simulink model "Template_v5_0_0_2026a_Linear"  (R2026a)
settings: Solver=ode4  StopTime=tsim  FixedStep=baseRate  RelTol=1e-6  AbsTol=1e-6
PreLoadFcn:
  | spot.buses.define;
  | if ~exist('simMode', 'var'), simMode = 1; end
InitFcn:
  | spot.buses.define;
  | if ~exist('simMode', 'var'), simMode = 1; end
values from neighbouring files (symbols this model uses):
  customControllerParamsBLACK = struct('unused', 0)    [SPOT_User_Parameters.m]
  customControllerParamsBLUE = struct('unused', 0)    [SPOT_User_Parameters.m]
  customControllerParamsRED = struct('unused', 0)    [SPOT_User_Parameters.m]
  customPlannerParamsBLACK = struct('unused', 0)    [SPOT_User_Parameters.m]
  customPlannerParamsBLUE = struct('unused', 0)    [SPOT_User_Parameters.m]
  customPlannerParamsRED = struct('unused', 0)    [SPOT_User_Parameters.m]
undefined symbols (not defined in the file or in its folder): baseRate, BLACK, BLUE, dataRate, DiscIntNeverNeededParam, F_thrusters_BLACK, F_thrusters_BLUE, F_thrusters_RED, home_states_BLACK, home_states_BLUE, home_states_RED, IBLACK, IBLUE, init_states_BLACK, init_states_BLUE, init_states_RED, IRED, K_BLACK, K_BLUE, K_RED, mBLACK, mBLUE, mRED, phase, Phase0_End, Phase1_End, Phase2_End, Phase3_End, Phase4_End, Phase5_End, PWMFreq, RED, tableDamping_BLACK, tableDamping_BLUE, tableDamping_RED, tableSlope, thrust_decay_BLACK, thrust_decay_BLUE, thrust_decay_RED, thruster_dist2CG_BLACK, thruster_dist2CG_BLUE, thruster_dist2CG_RED, time, xLength, yLength
libraries: nvidiaCommlib x1
(part 1 of 2)
settings Model: Creator=SPOT  LastModifiedBy=alexandercrain
settings OptimizationCC: MaxStackSize=200000
settings HardwareCC: ProdBitPerLong=64.0  ProdLargestAtomicInteger=LongLong  ProdLargestAtomicFloat=Double  ProdHWDeviceType=ARM Compatible->ARM Cortex-A (64-bit)
settings RTWCC: SystemTargetFile=ert.tlc  HardwareBoard=NVIDIA Jetson  TLCOptions="-aInlineSetEventsForThisBaseRateFcn=TLC_FALSE -aSuppressMultiTaskScheduler=TLC_FALSE  -aRateBasedStepFcn=0"  TargetLang=C++  Description=Embedded Coder
settings ERTTargetCC: ExtModeTransport=2.0  DynamicArrayContainerType=coder::array  SupportContinuousTime=on  SupportVariableSizeSignals=on
settings SimscapeCC: SimscapeNominalValues="[{\"value\":\"1\",\"unit\":\"A\"},{\"value\":\"1\",\"unit\":\"bar\"},{\"value\":\"1\",\"unit\":\"cm^2\"},{\"value\":\"1\",\"unit\":\"cm^3/s\"},{\"value\":\"1\",\"unit\":\"kJ/kg\"},{\"value\":\"1\",\"unit\":\"kW\"},{\"value\":\"1\",\"unit\":\"l\"},{\"value\":\"1\",\"unit\":\"N\"},{\"value\":\"1\",\"unit\":\"N*m\"},{\"value\":\"1\",\"unit\":\"V\"}]"  SimscapeLogType=none  SimscapeLogDataHistory=5000.0

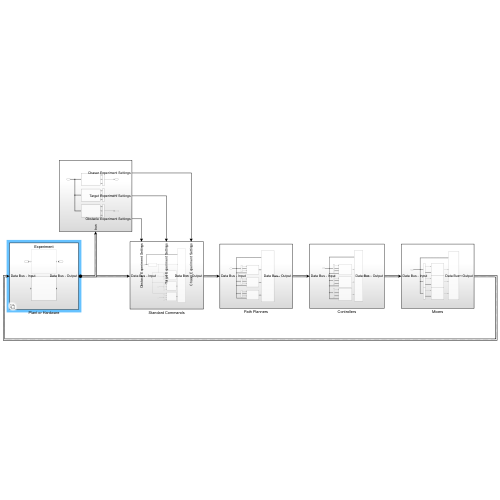
[thumbnail: Simulink's stored preview of the top-level diagram]
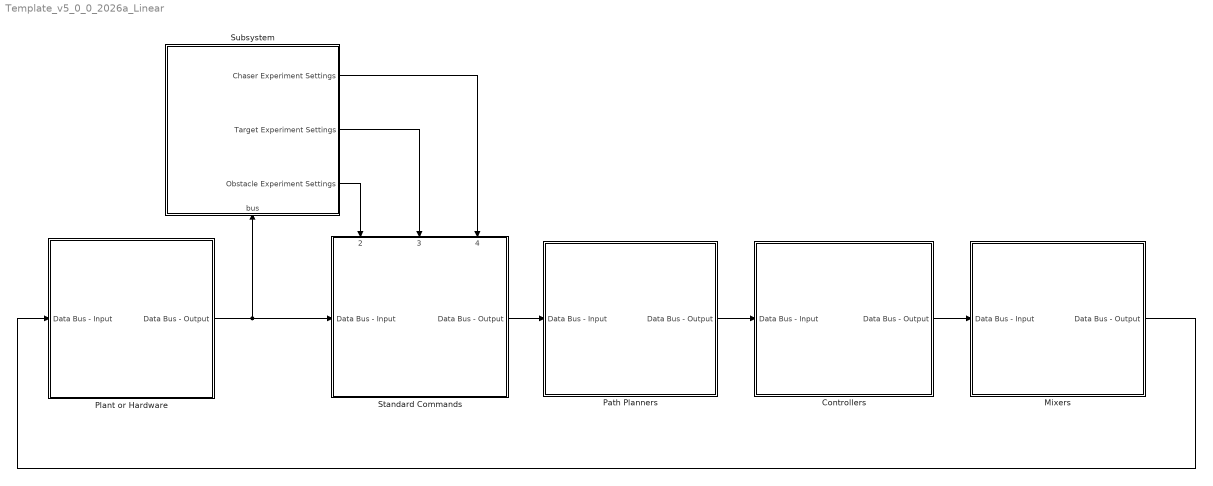
== system Template_v5_0_0_2026a_Linear ==
  Controllers : Subsystem
  Mixers : Subsystem
  Path Planners : Subsystem
  Plant or Hardware : Subsystem  Variant=on
  Standard Commands : Subsystem
      settings: PortSchema="{\"entries\":[{\"content\":{\"sides\":[{\"content\":{\"connectorIds\":[\"In1\"]},\"type\":\"ConnectorPlacement.EquallySpacedRectSide\",\"uuid\":\"35410a40-2c60-43fd-b064-79213576ed15\"},{\"content\":{\"connectorIds\":[\"Out1\"],\"side\":\"RIGHT\"},\"type\":\"ConnectorPlacement.EquallySpacedRectSide\",\"uuid\":\"393452b1-0693-434c-a64d-f21c96477400\"},{\"content\":{\"connectorIds\":[\"In2\",\"In3\",\"In4\"],\"side\":\"TOP\"},\"type\":\"ConnectorPlacement.EquallySpacedRectSide\",\"uuid\":\"b58be7cb-bf37-4612-971a-2054817b9ba4\"}]},\"type\":\"ConnectorPlacement.EquallySpacedConnector\",\"uuid\":\"cc986e65-98fa-43c9-b0c9-e9ff3e868710\"}],\"packageUris\":[\"http://schema.mathworks.com/mf0/Connector/R2020b\"],\"version\":\"1.0\"}"
  Subsystem : Subsystem
      settings: PortSchema="{\"entries\":[{\"content\":{\"sides\":[{\"content\":{},\"type\":\"ConnectorPlacement.EquallySpacedRectSide\",\"uuid\":\"3090d7f9-dd57-46ab-859b-619e032fcf1c\"},{\"content\":{\"connectorIds\":[\"Out1\",\"Out2\",\"Out3\"],\"side\":\"RIGHT\"},\"type\":\"ConnectorPlacement.EquallySpacedRectSide\",\"uuid\":\"1117e6ec-3262-4fcf-b5fe-08b02e10350e\"},{\"content\":{\"side\":\"TOP\"},\"type\":\"ConnectorPlacement.EquallySpacedRectSide\",\"uuid\":\"04f55234-f904-4f76-beb8-0b46031da363\"},{\"content\":{\"connectorIds\":[\"In1\"],\"side\":\"BOTTOM\"},\"type\":\"ConnectorPlacement.EquallySpacedRectSide\",\"uuid\":\"23d719f6-9ee1-4138-a3cc-61c2603cab92\"}]},\"type\":\"ConnectorPlacement.EquallySpacedConnector\",\"uuid\":\"bfffa1a7-ac7c-4cf9-962a-343a4a46f1db\"}],\"packageUris\":[\"http://schema.mathworks.com/mf0/Connector/R2020b\"],\"version\":\"1.0\"}"
  wires:
  Standard Commands/1(Data Bus - Output) -> Path Planners/1(Data Bus - Input)
  Path Planners/1(Data Bus - Output) -> Controllers/1(Data Bus - Input)
  Controllers/1(Data Bus - Output) -> Mixers/1(Data Bus - Input)
  Subsystem/1(Chaser Experiment Settings) -> Standard Commands/4(Chaser Experiment Settings)
  Subsystem/2(Target Experiment Settings) -> Standard Commands/3(Target Experiment Settings)
  Subsystem/3(Obstacle Experiment Settings) -> Standard Commands/2(Obstacle Experiment Settings)
  Mixers/1(Data Bus - Output) -> Plant or Hardware/1(Data Bus - Input)
  Plant or Hardware/1(Data Bus - Output) -> Standard Commands/1(Data Bus - Input), Subsystem/1(bus)

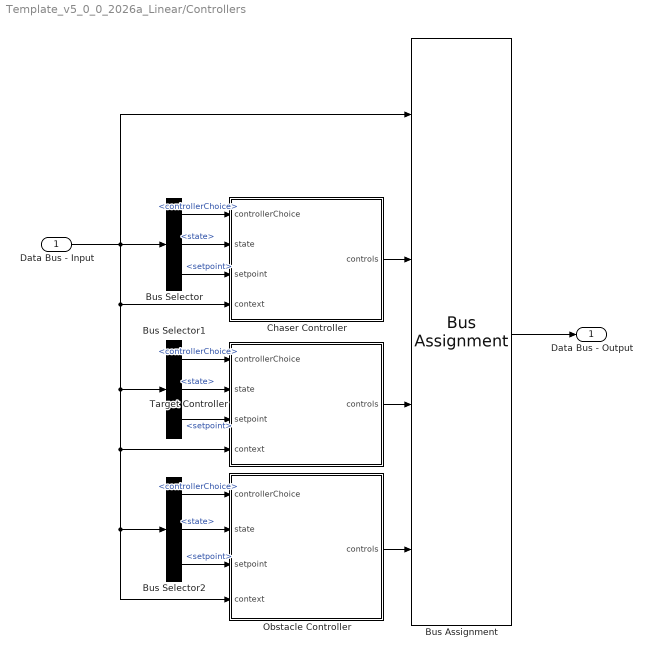
== system Template_v5_0_0_2026a_Linear/Controllers ==
  Data Bus - Input : Inport  OutDataTypeStr=Bus: SpotBus
  Bus Assignment : BusAssignment  AssignedSignals=RED.controls,BLACK.controls,BLUE.controls
  Bus Selector : BusSelector  OutputSignals=RED.command.controllerChoice,RED.state,RED.setpoint
  Bus Selector1 : BusSelector  OutputSignals=BLACK.command.controllerChoice,BLACK.state,BLACK.setpoint
  Bus Selector2 : BusSelector  OutputSignals=BLUE.command.controllerChoice,BLUE.state,BLUE.setpoint
  Chaser Controller : Subsystem  mask{K=K_RED, customParams=customControllerParamsRED}
      mask prompts: K "LQR Gain Matrix"; customParams "Custom Parameters Struct"
  Obstacle Controller : Subsystem  mask{K=K_BLUE, customParams=customControllerParamsBLUE}
      mask prompts: K "LQR Gain Matrix"; customParams "Custom Parameters Struct"
  Target Controller : Subsystem  mask{K=K_BLACK, customParams=customControllerParamsBLACK}
      mask prompts: K "LQR Gain Matrix"; customParams "Custom Parameters Struct"
  Data Bus - Output : Outport  OutDataTypeStr=Bus: SpotBus
  wires:
  Data Bus - Input/1 -> Bus Assignment/1, Target Controller/4(context), Obstacle Controller/4(context), Bus Selector2/1, Bus Selector1/1, Chaser Controller/4(context), Bus Selector/1
  Bus Selector/1 -> Chaser Controller/1(controllerChoice)  "<controllerChoice>"
  Bus Selector1/1 -> Target Controller/1(controllerChoice)  "<controllerChoice>"
  Bus Selector1/2 -> Target Controller/2(state)  "<state>"
  Bus Selector1/3 -> Target Controller/3(setpoint)  "<setpoint>"
  Bus Selector/2 -> Chaser Controller/2(state)  "<state>"
  Bus Selector/3 -> Chaser Controller/3(setpoint)  "<setpoint>"
  Bus Selector2/1 -> Obstacle Controller/1(controllerChoice)  "<controllerChoice>"
  Bus Selector2/2 -> Obstacle Controller/2(state)  "<state>"
  Bus Selector2/3 -> Obstacle Controller/3(setpoint)  "<setpoint>"
  Chaser Controller/1(controls) -> Bus Assignment/2
  Target Controller/1(controls) -> Bus Assignment/3
  Obstacle Controller/1(controls) -> Bus Assignment/4
  Bus Assignment/1 -> Data Bus - Output/1

== system Template_v5_0_0_2026a_Linear/Mixers ==
  Data Bus - Input : Inport  OutDataTypeStr=Bus: SpotBus
  Bus Assignment : BusAssignment  AssignedSignals=RED.duty,BLACK.duty,BLUE.duty
  Bus Selector : BusSelector  OutputSignals=RED.controls,RED.state
  Bus Selector1 : BusSelector  OutputSignals=BLACK.controls,BLACK.state
  Bus Selector2 : BusSelector  OutputSignals=BLUE.controls,BLUE.state
  Chaser Mixer : Subsystem  mask{thrusterDist=thruster_dist2CG_RED, thrust=F_thrusters_RED, decayPerValve=thrust_decay_RED}
      mask prompts: thrusterDist "Thruster Distances from CG"; thrust "Nominal Force per Thruster"; decayPerValve "Decay per Thruster"
  Obstacle Mixer : Subsystem  mask{thrusterDist=thruster_dist2CG_BLUE, thrust=F_thrusters_BLUE, decayPerValve=thrust_decay_BLUE}
      mask prompts: thrusterDist "Thruster Distances from CG"; thrust "Nominal Force per Thruster"; decayPerValve "Decay per Thruster"
  Target Mixer : Subsystem  mask{thrusterDist=thruster_dist2CG_BLACK, thrust=F_thrusters_BLACK, decayPerValve=thrust_decay_BLACK}
      mask prompts: thrusterDist "Thruster Distances from CG"; thrust "Nominal Force per Thruster"; decayPerValve "Decay per Thruster"
  Data Bus - Output : Outport  OutDataTypeStr=Bus: SpotBus
  wires:
  Data Bus - Input/1 -> Bus Selector2/1, Bus Selector1/1, Bus Assignment/1, Bus Selector/1
  Bus Selector/1 -> Chaser Mixer/1(controls)  "<controls>"
  Bus Selector/2 -> Chaser Mixer/2(state)  "<state>"
  Bus Selector2/1 -> Obstacle Mixer/1(controls)  "<controls>"
  Bus Selector1/1 -> Target Mixer/1(controls)  "<controls>"
  Bus Selector1/2 -> Target Mixer/2(state)  "<state>"
  Bus Selector2/2 -> Obstacle Mixer/2(state)  "<state>"
  Bus Assignment/1 -> Data Bus - Output/1
  Chaser Mixer/1(duty) -> Bus Assignment/2
  Target Mixer/1(duty) -> Bus Assignment/3
  Obstacle Mixer/1(duty) -> Bus Assignment/4

== system Template_v5_0_0_2026a_Linear/Path Planners ==
  Data Bus - Input : Inport  OutDataTypeStr=Bus: SpotBus
  Bus Assignment : BusAssignment  AssignedSignals=RED.setpoint,BLACK.setpoint,BLUE.setpoint
  Bus Selector : BusSelector  OutputSignals=RED.command.plannerChoice,RED.state,RED.command.goal
  Bus Selector1 : BusSelector  OutputSignals=BLACK.command.plannerChoice,BLACK.state,BLACK.command.goal
  Bus Selector2 : BusSelector  OutputSignals=BLUE.command.plannerChoice,BLUE.state,BLUE.command.goal
  Chaser Planner : Subsystem  mask{maxSpeed=0.05, maxTurnRate=0.09, horizon=2, customParams=customPlannerParamsRED, initialPose=init_states_RED}
      mask prompts: maxSpeed "Cruising Speed"; maxTurnRate "Cruising Turn Rate"; horizon "Setpoint Distance"; customParams "User Parameters"; initialPose "Initial Pose"
  Obstacle Planner : Subsystem  mask{maxSpeed=0.05, maxTurnRate=0.09, horizon=2, customParams=customPlannerParamsBLUE, initialPose=init_states_BLUE}
      mask prompts: maxSpeed "Cruising Speed"; maxTurnRate "Cruising Turn Rate"; horizon "Setpoint Distance"; customParams "User Parameters"; initialPose "Initial Pose"
  Target Planner : Subsystem  mask{maxSpeed=0.05, maxTurnRate=0.09, horizon=2, customParams=customPlannerParamsBLACK, initialPose=init_states_BLACK}
      mask prompts: maxSpeed "Cruising Speed"; maxTurnRate "Cruising Turn Rate"; horizon "Setpoint Distance"; customParams "User Parameters"; initialPose "Initial Pose"
  Data Bus - Output : Outport  OutDataTypeStr=Bus: SpotBus
  wires:
  Data Bus - Input/1 -> Chaser Planner/4(context), Target Planner/4(context), Obstacle Planner/4(context), Bus Selector2/1, Bus Selector1/1, Bus Assignment/1, Bus Selector/1
  Chaser Planner/1(setpoint) -> Bus Assignment/2
  Target Planner/1(setpoint) -> Bus Assignment/3
  Obstacle Planner/1(setpoint) -> Bus Assignment/4
  Bus Assignment/1 -> Data Bus - Output/1
  Bus Selector/3 -> Chaser Planner/3(goal)  "<goal>"
  Bus Selector/2 -> Chaser Planner/2(state)  "<state>"
  Bus Selector/1 -> Chaser Planner/1(plannerChoice)  "<plannerChoice>"
  Bus Selector1/1 -> Target Planner/1(plannerChoice)  "<plannerChoice>"
  Bus Selector1/2 -> Target Planner/2(state)  "<state>"
  Bus Selector1/3 -> Target Planner/3(goal)  "<goal>"
  Bus Selector2/1 -> Obstacle Planner/1(plannerChoice)  "<plannerChoice>"
  Bus Selector2/2 -> Obstacle Planner/2(state)  "<state>"
  Bus Selector2/3 -> Obstacle Planner/3(goal)  "<goal>"

== system Template_v5_0_0_2026a_Linear/Plant or Hardware ==
  Data Bus - Input : Inport
  Experiment : Subsystem  VariantControl=simMode == 0
  Simulation : Subsystem  VariantControl=simMode == 1
  Data Bus - Output : Outport

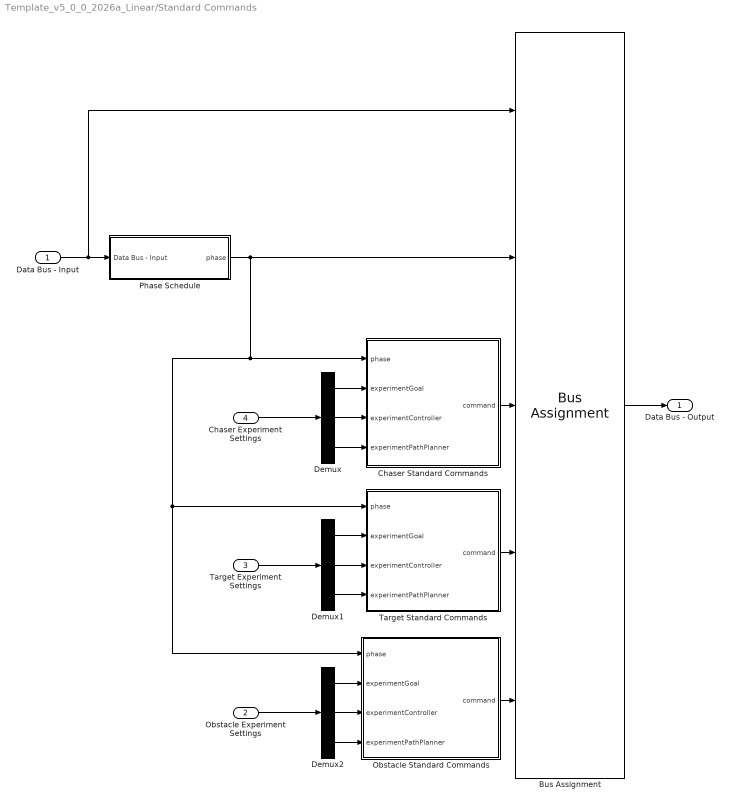
== system Template_v5_0_0_2026a_Linear/Standard Commands ==
  Data Bus - Input : Inport  OutDataTypeStr=Bus: SpotBus
  Obstacle Experiment Settings : Inport  Port=2
  Target Experiment Settings : Inport  Port=3
  Chaser Experiment Settings : Inport  Port=4
  Bus Assignment : BusAssignment  AssignedSignals=phase,RED.command,BLACK.command,BLUE.command
  Chaser Standard Commands : Subsystem  mask{initialPose=init_states_RED, homePose=home_states_RED}
      mask prompts: initialPose "Initial Pose"; homePose "Home Pose"
  Demux : Demux  Outputs=[3,1,1]
  Demux1 : Demux  Outputs=[3,1,1]
  Demux2 : Demux  Outputs=[3,1,1]
  Obstacle Standard Commands : Subsystem  mask{initialPose=init_states_BLUE, homePose=home_states_BLUE}
      mask prompts: initialPose "Initial Pose"; homePose "Home Pose"
  Phase Schedule : Subsystem
  Target Standard Commands : Subsystem  mask{initialPose=init_states_BLACK, homePose=home_states_BLACK}
      mask prompts: initialPose "Initial Pose"; homePose "Home Pose"
  Data Bus - Output : Outport  OutDataTypeStr=Bus: SpotBus
  wires:
  Phase Schedule/1(phase) -> Bus Assignment/2, Chaser Standard Commands/1(phase), Target Standard Commands/1(phase), Obstacle Standard Commands/1(phase)
  Data Bus - Input/1 -> Bus Assignment/1, Phase Schedule/1(Data Bus - Input)
  Chaser Standard Commands/1(command) -> Bus Assignment/3
  Target Standard Commands/1(command) -> Bus Assignment/4
  Obstacle Standard Commands/1(command) -> Bus Assignment/5
  Bus Assignment/1 -> Data Bus - Output/1
  Demux/1 -> Chaser Standard Commands/2(experimentGoal)
  Demux/2 -> Chaser Standard Commands/3(experimentController)
  Demux/3 -> Chaser Standard Commands/4(experimentPathPlanner)
  Chaser Experiment Settings/1 -> Demux/1
  Demux1/1 -> Target Standard Commands/2(experimentGoal)
  Demux1/2 -> Target Standard Commands/3(experimentController)
  Demux1/3 -> Target Standard Commands/4(experimentPathPlanner)
  Target Experiment Settings/1 -> Demux1/1
  Demux2/1 -> Obstacle Standard Commands/2(experimentGoal)
  Demux2/2 -> Obstacle Standard Commands/3(experimentController)
  Demux2/3 -> Obstacle Standard Commands/4(experimentPathPlanner)
  Obstacle Experiment Settings/1 -> Demux2/1

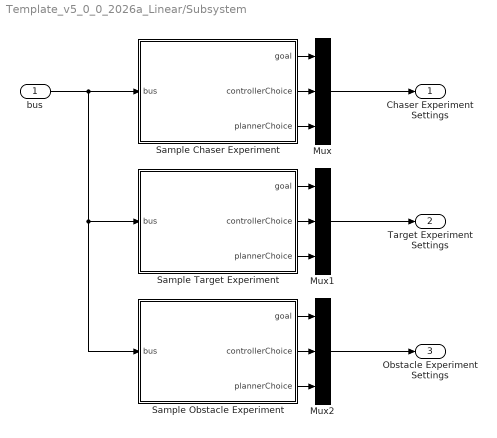
== system Template_v5_0_0_2026a_Linear/Subsystem ==
  bus : Inport  OutDataTypeStr=Bus: SpotBus
  Mux : Mux  Inputs=3
  Mux1 : Mux  Inputs=3
  Mux2 : Mux  Inputs=3
  Sample Chaser Experiment : MATLAB Function  TreatAsAtomicUnit=on
  Sample Obstacle Experiment : MATLAB Function  TreatAsAtomicUnit=on
  Sample Target Experiment : MATLAB Function  TreatAsAtomicUnit=on
  Chaser Experiment Settings : Outport
  Target Experiment Settings : Outport  Port=2
  Obstacle Experiment Settings : Outport  Port=3
  wires:
  bus/1 -> Sample Obstacle Experiment/1(bus), Sample Target Experiment/1(bus), Sample Chaser Experiment/1(bus)
  Sample Chaser Experiment/1(goal) -> Mux/1
  Sample Chaser Experiment/2(controllerChoice) -> Mux/2
  Sample Chaser Experiment/3(plannerChoice) -> Mux/3
  Sample Target Experiment/1(goal) -> Mux1/1
  Sample Target Experiment/2(controllerChoice) -> Mux1/2
  Sample Target Experiment/3(plannerChoice) -> Mux1/3
  Sample Obstacle Experiment/1(goal) -> Mux2/1
  Sample Obstacle Experiment/2(controllerChoice) -> Mux2/2
  Sample Obstacle Experiment/3(plannerChoice) -> Mux2/3
  Mux/1 -> Chaser Experiment Settings/1
  Mux1/1 -> Target Experiment Settings/1
  Mux2/1 -> Obstacle Experiment Settings/1

== system Template_v5_0_0_2026a_Linear/Controllers/Chaser Controller ==
  controllerChoice : Inport
  state : Inport  Port=2
  setpoint : Inport  Port=3
  context : Inport  Port=4
  callController : MATLAB Function  TreatAsAtomicUnit=on
  controls : Outport
  wires:
  callController/1(controls) -> controls/1
  controllerChoice/1 -> callController/1(controllerChoice)
  state/1 -> callController/2(state)
  setpoint/1 -> callController/3(setpoint)
  context/1 -> callController/4(context)

== system Template_v5_0_0_2026a_Linear/Controllers/Obstacle Controller ==
  controllerChoice : Inport
  state : Inport  Port=2
  setpoint : Inport  Port=3
  context : Inport  Port=4
  callController : MATLAB Function  TreatAsAtomicUnit=on
  controls : Outport
  wires:
  setpoint/1 -> callController/3(setpoint)
  callController/1(controls) -> controls/1
  controllerChoice/1 -> callController/1(controllerChoice)
  context/1 -> callController/4(context)
  state/1 -> callController/2(state)

== system Template_v5_0_0_2026a_Linear/Controllers/Target Controller ==
  controllerChoice : Inport
  state : Inport  Port=2
  setpoint : Inport  Port=3
  context : Inport  Port=4
  callController : MATLAB Function  TreatAsAtomicUnit=on
  controls : Outport
  wires:
  setpoint/1 -> callController/3(setpoint)
  callController/1(controls) -> controls/1
  controllerChoice/1 -> callController/1(controllerChoice)
  context/1 -> callController/4(context)
  state/1 -> callController/2(state)

== system Template_v5_0_0_2026a_Linear/Mixers/Chaser Mixer ==
  controls : Inport
  state : Inport  Port=2
  callMixer : MATLAB Function  TreatAsAtomicUnit=on
  duty : Outport
  wires:
  controls/1 -> callMixer/1(controls)
  state/1 -> callMixer/2(state)
  callMixer/1(duty) -> duty/1

== system Template_v5_0_0_2026a_Linear/Mixers/Obstacle Mixer ==
  controls : Inport
  state : Inport  Port=2
  callMixer : MATLAB Function  TreatAsAtomicUnit=on
  duty : Outport
  wires:
  state/1 -> callMixer/2(state)
  controls/1 -> callMixer/1(controls)
  callMixer/1(duty) -> duty/1

== system Template_v5_0_0_2026a_Linear/Mixers/Target Mixer ==
  controls : Inport
  state : Inport  Port=2
  callMixer : MATLAB Function  TreatAsAtomicUnit=on
  duty : Outport
  wires:
  state/1 -> callMixer/2(state)
  controls/1 -> callMixer/1(controls)
  callMixer/1(duty) -> duty/1

== system Template_v5_0_0_2026a_Linear/Path Planners/Chaser Planner ==
  plannerChoice : Inport
  state : Inport  Port=2
  goal : Inport  Port=3
  context : Inport  Port=4
  Unit Delay : UnitDelay  InitialCondition=initialPose  SampleTime=-1
  callPlanner : MATLAB Function  TreatAsAtomicUnit=on
  setpoint : Outport
  wires:
  state/1 -> callPlanner/2(state)
  callPlanner/1(setpoint) -> setpoint/1
  goal/1 -> Unit Delay/1, callPlanner/3(goal)
  plannerChoice/1 -> callPlanner/1(plannerChoice)
  context/1 -> callPlanner/5(context)
  Unit Delay/1 -> callPlanner/4(previousGoal)

== system Template_v5_0_0_2026a_Linear/Path Planners/Obstacle Planner ==
  plannerChoice : Inport
  state : Inport  Port=2
  goal : Inport  Port=3
  context : Inport  Port=4
  Unit Delay : UnitDelay  InitialCondition=initialPose  SampleTime=-1
  callPlanner : MATLAB Function  TreatAsAtomicUnit=on
  setpoint : Outport
  wires:
  callPlanner/1(setpoint) -> setpoint/1
  Unit Delay/1 -> callPlanner/4(previousGoal)
  context/1 -> callPlanner/5(context)
  goal/1 -> Unit Delay/1, callPlanner/3(goal)
  plannerChoice/1 -> callPlanner/1(plannerChoice)
  state/1 -> callPlanner/2(state)

== system Template_v5_0_0_2026a_Linear/Path Planners/Target Planner ==
  plannerChoice : Inport
  state : Inport  Port=2
  goal : Inport  Port=3
  context : Inport  Port=4
  Unit Delay : UnitDelay  InitialCondition=initialPose  SampleTime=-1
  callPlanner : MATLAB Function  TreatAsAtomicUnit=on
  setpoint : Outport
  wires:
  callPlanner/1(setpoint) -> setpoint/1
  Unit Delay/1 -> callPlanner/4(previousGoal)
  context/1 -> callPlanner/5(context)
  goal/1 -> Unit Delay/1, callPlanner/3(goal)
  plannerChoice/1 -> callPlanner/1(plannerChoice)
  state/1 -> callPlanner/2(state)

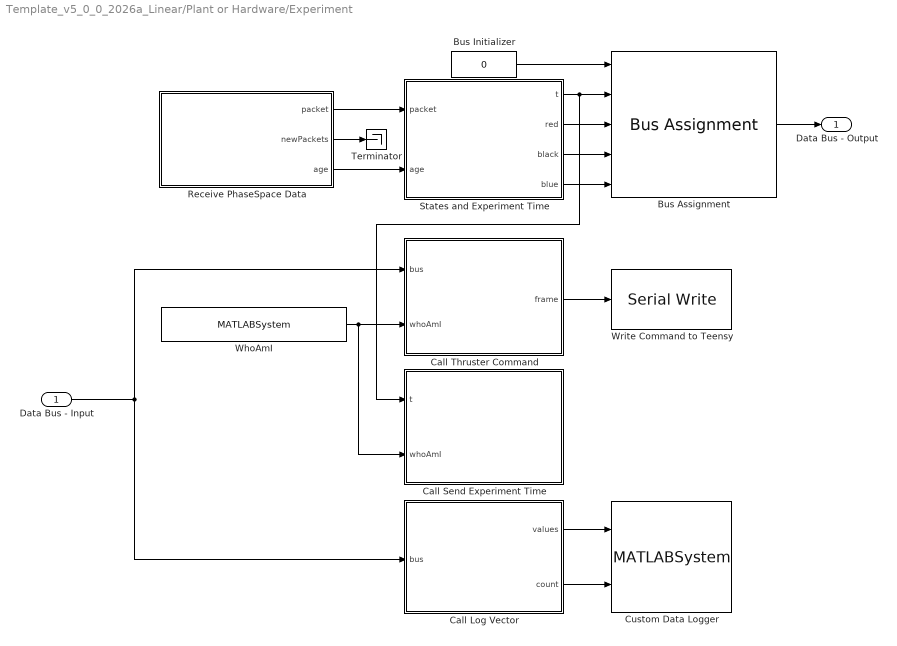
== system Template_v5_0_0_2026a_Linear/Plant or Hardware/Experiment ==
  Data Bus - Input : Inport  OutDataTypeStr=Bus: SpotBus
  Bus Assignment : BusAssignment  AssignedSignals=time,RED.state,BLACK.state,BLUE.state
  Bus Initializer : Constant  Value=0  OutDataTypeStr=Bus: SpotBus
  Call Log Vector : MATLAB Function  TreatAsAtomicUnit=on
  Call Send Experiment Time : MATLAB Function  TreatAsAtomicUnit=on
  Call Thruster Command : MATLAB Function  TreatAsAtomicUnit=on
  Custom Data Logger : MATLABSystem  System=spot.hardware.CustomDataLogger
      mask Type: spot.hardware.CustomDataLogger
  Receive PhaseSpace Data : MATLAB Function  TreatAsAtomicUnit=on  SystemSampleTime=baseRate
  States and Experiment Time : MATLAB Function  TreatAsAtomicUnit=on
  Terminator : Terminator
  WhoAmI : MATLABSystem  System=spot.hardware.IdentifyPlatform  SampleTime=baseRate
      mask Type: spot.hardware.IdentifyPlatform
  Write Command to Teensy : nvidiaCommlib/Serial Write  SCIModule=/dev/ttyACM0  Baudrate_=115200  Parity=None  StopBits_=1
  Data Bus - Output : Outport  OutDataTypeStr=Bus: SpotBus
  wires:
  Receive PhaseSpace Data/2(newPackets) -> Terminator/1
  Receive PhaseSpace Data/1(packet) -> States and Experiment Time/1(packet)
  Receive PhaseSpace Data/3(age) -> States and Experiment Time/2(age)
  Bus Initializer/1 -> Bus Assignment/1
  States and Experiment Time/1(t) -> Bus Assignment/2, Call Send Experiment Time/1(t)
  States and Experiment Time/2(red) -> Bus Assignment/3
  States and Experiment Time/3(black) -> Bus Assignment/4
  States and Experiment Time/4(blue) -> Bus Assignment/5
  Bus Assignment/1 -> Data Bus - Output/1
  Call Thruster Command/1(frame) -> Write Command to Teensy/1
  Call Log Vector/1(values) -> Custom Data Logger/1
  Call Log Vector/2(count) -> Custom Data Logger/2
  WhoAmI/1 -> Call Send Experiment Time/2(whoAmI), Call Thruster Command/2(whoAmI)
  Data Bus - Input/1 -> Call Thruster Command/1(bus), Call Log Vector/1(bus)

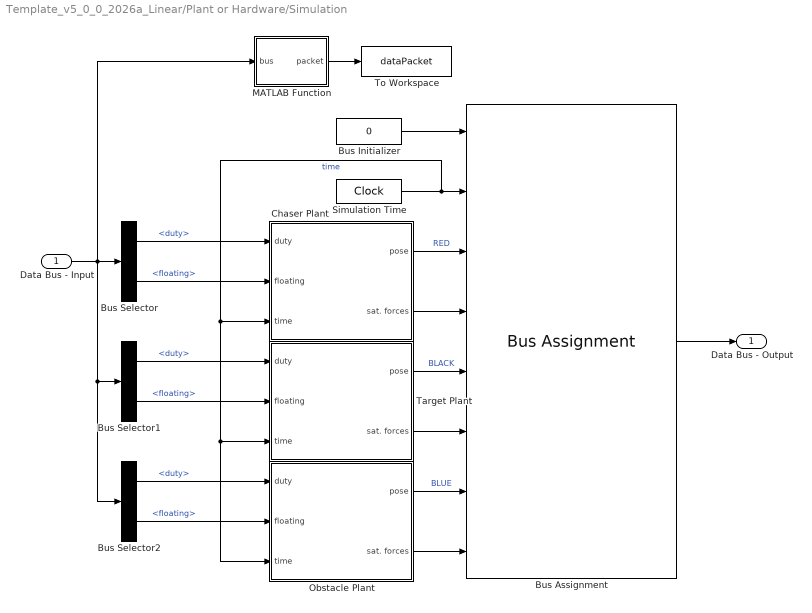
== system Template_v5_0_0_2026a_Linear/Plant or Hardware/Simulation ==
  Data Bus - Input : Inport  OutDataTypeStr=Bus: SpotBus
  Bus Assignment : BusAssignment  AssignedSignals=time,RED.state,RED.satForces,BLACK.state,BLACK.satForces,BLUE.state,BLUE.satForces
  Bus Selector : BusSelector  OutputSignals=RED.duty,RED.command.floating
  Bus Selector1 : BusSelector  OutputSignals=BLACK.duty,BLACK.command.floating
  Bus Selector2 : BusSelector  OutputSignals=BLUE.duty,BLUE.command.floating
  Bus Initializer : Constant  Value=0  OutDataTypeStr=Bus: SpotBus
  Chaser Plant : Subsystem  mask{mass=mRED, inertia=IRED, tableDamping=tableDamping_RED, initialPose=init_states_RED, decayPerValve=thrust_decay_RED, thrust=F_thrusters_RED, thrusterDist=thruster_dist2CG_RED}
      mask prompts: mass "Mass [kg]"; inertia "Inertia [kg.m^2]"; tableDamping "Table Damping [1/s]"; initialPose "Initial Pose [m, m, rad]"; decayPerValve "Decay per Thruster"; thrust "Nominal Thruster Force"; thrusterDist "Thruster Distances"
      mask DialogControl DescTextVar Prompt: Calculates the acceleration for a rigid-body on a sloped near-frictionless granite table.
  MATLAB Function : MATLAB Function  TreatAsAtomicUnit=on
  Obstacle Plant : Subsystem  mask{mass=mBLUE, inertia=IBLUE, tableDamping=tableDamping_BLUE, initialPose=init_states_BLUE, decayPerValve=thrust_decay_BLUE, thrust=F_thrusters_BLUE, thrusterDist=thruster_dist2CG_BLUE}
      mask prompts: mass "Mass [kg]"; inertia "Inertia [kg.m^2]"; tableDamping "Table Damping [1/s]"; initialPose "Initial Pose [m, m, rad]"; decayPerValve "Decay per Thruster"; thrust "Nominal Thruster Force"; thrusterDist "Thruster Distances"
      mask DialogControl DescTextVar Prompt: Calculates the acceleration for a rigid-body on a sloped near-frictionless granite table.
  Simulation Time : DigitalClock  SampleTime=baseRate
  Target Plant : Subsystem  mask{mass=mBLACK, inertia=IBLACK, tableDamping=tableDamping_BLACK, initialPose=init_states_BLACK, decayPerValve=thrust_decay_BLACK, thrust=F_thrusters_BLACK, thrusterDist=thruster_dist2CG_BLACK}
      mask prompts: mass "Mass [kg]"; inertia "Inertia [kg.m^2]"; tableDamping "Table Damping [1/s]"; initialPose "Initial Pose [m, m, rad]"; decayPerValve "Decay per Thruster"; thrust "Nominal Thruster Force"; thrusterDist "Thruster Distances"
      mask DialogControl DescTextVar Prompt: Calculates the acceleration for a rigid-body on a sloped near-frictionless granite table.
  To Workspace : ToWorkspace  VariableName=dataPacket  SaveFormat=Timeseries  SampleTime=-1
  Data Bus - Output : Outport  OutDataTypeStr=Bus: SpotBus
  wires:
  Bus Selector/2 -> Chaser Plant/2(floating)  "<floating>"
  Bus Initializer/1 -> Bus Assignment/1
  Chaser Plant/1(pose) -> Bus Assignment/3  "RED"
  Obstacle Plant/1(pose) -> Bus Assignment/7  "BLUE"
  Target Plant/1(pose) -> Bus Assignment/5  "BLACK"
  Simulation Time/1 -> Obstacle Plant/3(time), Target Plant/3(time), Chaser Plant/3(time), Bus Assignment/2  "time"
  Bus Assignment/1 -> Data Bus - Output/1
  Bus Selector1/2 -> Target Plant/2(floating)  "<floating>"
  Bus Selector2/2 -> Obstacle Plant/2(floating)  "<floating>"
  Bus Selector/1 -> Chaser Plant/1(duty)  "<duty>"
  Bus Selector1/1 -> Target Plant/1(duty)  "<duty>"
  Bus Selector2/1 -> Obstacle Plant/1(duty)  "<duty>"
  Chaser Plant/2(sat. forces) -> Bus Assignment/4
  Target Plant/2(sat. forces) -> Bus Assignment/6
  Obstacle Plant/2(sat. forces) -> Bus Assignment/8
  Data Bus - Input/1 -> MATLAB Function/1(bus), Bus Selector2/1, Bus Selector1/1, Bus Selector/1
  MATLAB Function/1(packet) -> To Workspace/1

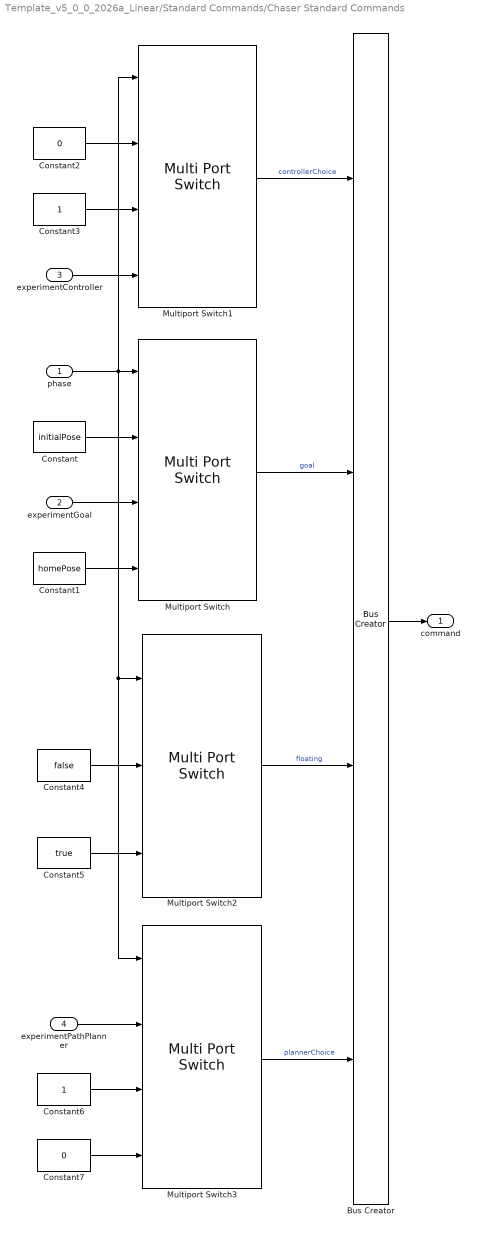
== system Template_v5_0_0_2026a_Linear/Standard Commands/Chaser Standard Commands ==
  phase : Inport
  experimentGoal : Inport  Port=2
  experimentController : Inport  Port=3
  experimentPathPlanner : Inport  Port=4
  Bus Creator : BusCreator  Inputs=4  OutDataTypeStr=Bus: PhaseCommand
  Constant : Constant  Value=initialPose
  Constant1 : Constant  Value=homePose
  Constant2 : Constant  Value=0
  Constant3 : Constant
  Constant4 : Constant  Value=false
  Constant5 : Constant  Value=true
  Constant6 : Constant
  Constant7 : Constant  Value=0
  Multiport Switch : MultiPortSwitch  DataPortOrder=Specify indices  DataPortIndices={[0 1 2], 3, [4 5 6]}  SaturateOnIntegerOverflow=off  InputSameDT=off
  Multiport Switch1 : MultiPortSwitch  DataPortOrder=Specify indices  DataPortIndices={[0 1 6], [2 4 5], 3}  SaturateOnIntegerOverflow=off  InputSameDT=off
  Multiport Switch2 : MultiPortSwitch  DataPortOrder=Specify indices  Inputs=2  DataPortIndices={[0 6], [1 2 3 4 5]}  SaturateOnIntegerOverflow=off  InputSameDT=off
  Multiport Switch3 : MultiPortSwitch  DataPortOrder=Specify indices  DataPortIndices={3, [2 4 5], [0 1 6]}  SaturateOnIntegerOverflow=off  InputSameDT=off
  command : Outport
  wires:
  phase/1 -> Multiport Switch3/1, Multiport Switch2/1, Multiport Switch1/1, Multiport Switch/1
  Constant/1 -> Multiport Switch/2
  experimentGoal/1 -> Multiport Switch/3
  Constant1/1 -> Multiport Switch/4
  Constant2/1 -> Multiport Switch1/2
  Constant3/1 -> Multiport Switch1/3
  experimentController/1 -> Multiport Switch1/4
  Constant4/1 -> Multiport Switch2/2
  Constant5/1 -> Multiport Switch2/3
  Bus Creator/1 -> command/1
  Multiport Switch1/1 -> Bus Creator/1  "controllerChoice"
  Multiport Switch/1 -> Bus Creator/2  "goal"
  Multiport Switch2/1 -> Bus Creator/3  "floating"
  experimentPathPlanner/1 -> Multiport Switch3/2
  Constant6/1 -> Multiport Switch3/3
  Constant7/1 -> Multiport Switch3/4
  Multiport Switch3/1 -> Bus Creator/4  "plannerChoice"

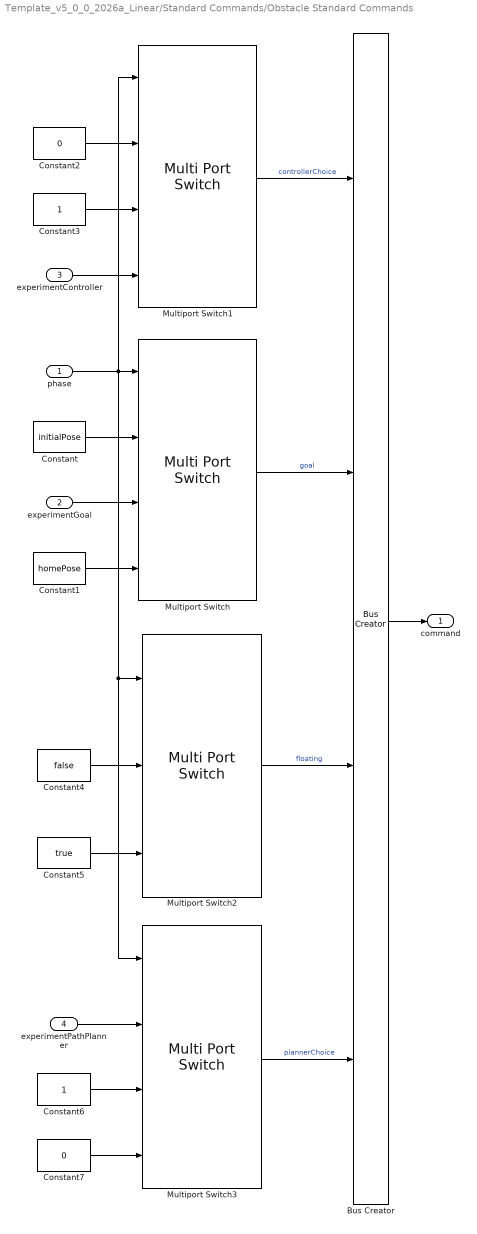
== system Template_v5_0_0_2026a_Linear/Standard Commands/Obstacle Standard Commands ==
  phase : Inport
  experimentGoal : Inport  Port=2
  experimentController : Inport  Port=3
  experimentPathPlanner : Inport  Port=4
  Bus Creator : BusCreator  Inputs=4  OutDataTypeStr=Bus: PhaseCommand
  Constant : Constant  Value=initialPose
  Constant1 : Constant  Value=homePose
  Constant2 : Constant  Value=0
  Constant3 : Constant
  Constant4 : Constant  Value=false
  Constant5 : Constant  Value=true
  Constant6 : Constant
  Constant7 : Constant  Value=0
  Multiport Switch : MultiPortSwitch  DataPortOrder=Specify indices  DataPortIndices={[0 1 2], 3, [4 5 6]}  SaturateOnIntegerOverflow=off  InputSameDT=off
  Multiport Switch1 : MultiPortSwitch  DataPortOrder=Specify indices  DataPortIndices={[0 1 6], [2 4 5], 3}  SaturateOnIntegerOverflow=off  InputSameDT=off
  Multiport Switch2 : MultiPortSwitch  DataPortOrder=Specify indices  Inputs=2  DataPortIndices={[0 6], [1 2 3 4 5]}  SaturateOnIntegerOverflow=off  InputSameDT=off
  Multiport Switch3 : MultiPortSwitch  DataPortOrder=Specify indices  DataPortIndices={3, [2 4 5], [0 1 6]}  SaturateOnIntegerOverflow=off  InputSameDT=off
  command : Outport
  wires:
  Constant3/1 -> Multiport Switch1/3
  Multiport Switch2/1 -> Bus Creator/3  "floating"
  Multiport Switch1/1 -> Bus Creator/1  "controllerChoice"
  Multiport Switch/1 -> Bus Creator/2  "goal"
  Multiport Switch3/1 -> Bus Creator/4  "plannerChoice"
  phase/1 -> Multiport Switch3/1, Multiport Switch2/1, Multiport Switch1/1, Multiport Switch/1
  Constant2/1 -> Multiport Switch1/2
  Bus Creator/1 -> command/1
  Constant6/1 -> Multiport Switch3/3
  Constant1/1 -> Multiport Switch/4
  experimentController/1 -> Multiport Switch1/4
  Constant5/1 -> Multiport Switch2/3
  Constant7/1 -> Multiport Switch3/4
  experimentGoal/1 -> Multiport Switch/3
  experimentPathPlanner/1 -> Multiport Switch3/2
  Constant4/1 -> Multiport Switch2/2
  Constant/1 -> Multiport Switch/2

== system Template_v5_0_0_2026a_Linear/Standard Commands/Phase Schedule ==
  Data Bus - Input : Inport  OutDataTypeStr=Bus: SpotBus
  Bus Selector : BusSelector  OutputSignals=time
  Phase End Times : Constant  Value=[Phase0_End Phase1_End Phase2_End Phase3_End Phase4_End Phase5_End]
  Relational Operator : RelationalOperator  OutDataTypeStr=boolean  RndMeth=Simplest  InputSameDT=off
  Sum : Sum  Inputs=+  OutDataTypeStr=double
  phase : Outport
  wires:
  Phase End Times/1 -> Relational Operator/2
  Relational Operator/1 -> Sum/1
  Sum/1 -> phase/1
  Data Bus - Input/1 -> Bus Selector/1
  Bus Selector/1 -> Relational Operator/1  "<time>"

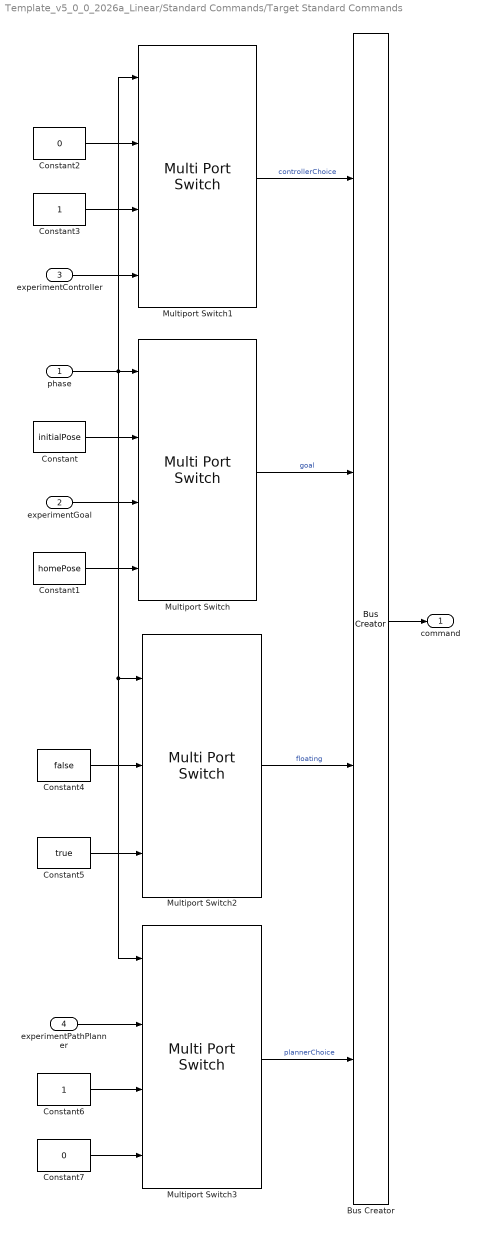
== system Template_v5_0_0_2026a_Linear/Standard Commands/Target Standard Commands ==
  phase : Inport
  experimentGoal : Inport  Port=2
  experimentController : Inport  Port=3
  experimentPathPlanner : Inport  Port=4
  Bus Creator : BusCreator  Inputs=4  OutDataTypeStr=Bus: PhaseCommand
  Constant : Constant  Value=initialPose
  Constant1 : Constant  Value=homePose
  Constant2 : Constant  Value=0
  Constant3 : Constant
  Constant4 : Constant  Value=false
  Constant5 : Constant  Value=true
  Constant6 : Constant
  Constant7 : Constant  Value=0
  Multiport Switch : MultiPortSwitch  DataPortOrder=Specify indices  DataPortIndices={[0 1 2], 3, [4 5 6]}  SaturateOnIntegerOverflow=off  InputSameDT=off
  Multiport Switch1 : MultiPortSwitch  DataPortOrder=Specify indices  DataPortIndices={[0 1 6], [2 4 5], 3}  SaturateOnIntegerOverflow=off  InputSameDT=off
  Multiport Switch2 : MultiPortSwitch  DataPortOrder=Specify indices  Inputs=2  DataPortIndices={[0 6], [1 2 3 4 5]}  SaturateOnIntegerOverflow=off  InputSameDT=off
  Multiport Switch3 : MultiPortSwitch  DataPortOrder=Specify indices  DataPortIndices={3, [2 4 5], [0 1 6]}  SaturateOnIntegerOverflow=off  InputSameDT=off
  command : Outport
  wires:
  Multiport Switch/1 -> Bus Creator/2  "goal"
  Constant3/1 -> Multiport Switch1/3
  experimentGoal/1 -> Multiport Switch/3
  Multiport Switch1/1 -> Bus Creator/1  "controllerChoice"
  Constant7/1 -> Multiport Switch3/4
  Constant4/1 -> Multiport Switch2/2
  Multiport Switch2/1 -> Bus Creator/3  "floating"
  Multiport Switch3/1 -> Bus Creator/4  "plannerChoice"
  Constant2/1 -> Multiport Switch1/2
  Constant5/1 -> Multiport Switch2/3
  phase/1 -> Multiport Switch3/1, Multiport Switch2/1, Multiport Switch1/1, Multiport Switch/1
  Bus Creator/1 -> command/1
  Constant/1 -> Multiport Switch/2
  Constant1/1 -> Multiport Switch/4
  experimentController/1 -> Multiport Switch1/4
  Constant6/1 -> Multiport Switch3/3
  experimentPathPlanner/1 -> Multiport Switch3/2

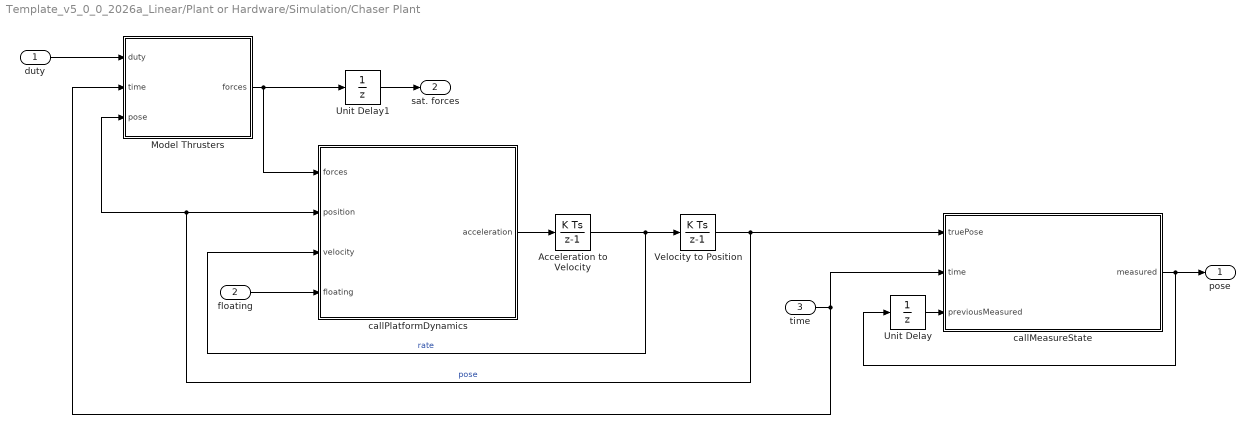
== system Template_v5_0_0_2026a_Linear/Plant or Hardware/Simulation/Chaser Plant ==
  duty : Inport
  floating : Inport  Port=2
  time : Inport  Port=3
  Acceleration to Velocity : DiscreteIntegrator  SampleTime=-1  ICPrevOutput=DiscIntNeverNeededParam  ICPrevScaledInput=DiscIntNeverNeededParam
  Model Thrusters : Subsystem
  Unit Delay : UnitDelay  SampleTime=-1
  Unit Delay1 : UnitDelay  SampleTime=-1
  Velocity to Position : DiscreteIntegrator  InitialCondition=initialPose  SampleTime=-1  ICPrevOutput=DiscIntNeverNeededParam  ICPrevScaledInput=DiscIntNeverNeededParam
  callMeasureState : MATLAB Function  TreatAsAtomicUnit=on
  callPlatformDynamics : MATLAB Function  TreatAsAtomicUnit=on
  pose : Outport
  sat. forces : Outport  Port=2
  wires:
  callPlatformDynamics/1(acceleration) -> Acceleration to Velocity/1
  callMeasureState/1(measured) -> Unit Delay/1, pose/1
  Acceleration to Velocity/1 -> callPlatformDynamics/3(velocity), Velocity to Position/1  "rate"
  floating/1 -> callPlatformDynamics/4(floating)
  Velocity to Position/1 -> callMeasureState/1(truePose), Model Thrusters/3(pose), callPlatformDynamics/2(position)  "pose"
  Unit Delay/1 -> callMeasureState/3(previousMeasured)
  time/1 -> callMeasureState/2(time), Model Thrusters/2(time)
  Unit Delay1/1 -> sat. forces/1
  duty/1 -> Model Thrusters/1(duty)
  Model Thrusters/1(forces) -> Unit Delay1/1, callPlatformDynamics/1(forces)

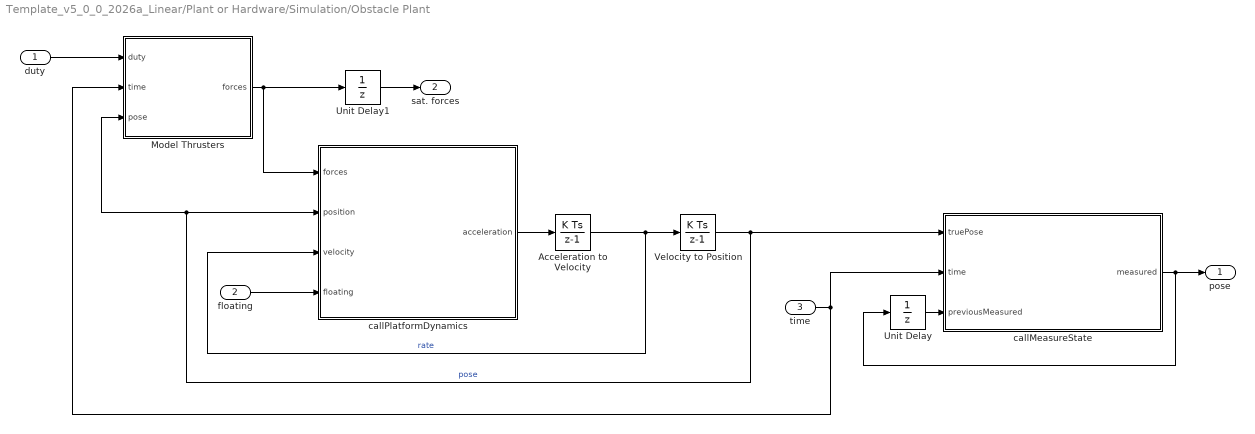
== system Template_v5_0_0_2026a_Linear/Plant or Hardware/Simulation/Obstacle Plant ==
  duty : Inport
  floating : Inport  Port=2
  time : Inport  Port=3
  Acceleration to Velocity : DiscreteIntegrator  SampleTime=-1  ICPrevOutput=DiscIntNeverNeededParam  ICPrevScaledInput=DiscIntNeverNeededParam
  Model Thrusters : Subsystem
  Unit Delay : UnitDelay  SampleTime=-1
  Unit Delay1 : UnitDelay  SampleTime=-1
  Velocity to Position : DiscreteIntegrator  InitialCondition=initialPose  SampleTime=-1  ICPrevOutput=DiscIntNeverNeededParam  ICPrevScaledInput=DiscIntNeverNeededParam
  callMeasureState : MATLAB Function  TreatAsAtomicUnit=on
  callPlatformDynamics : MATLAB Function  TreatAsAtomicUnit=on
  pose : Outport
  sat. forces : Outport  Port=2
  wires:
  callMeasureState/1(measured) -> Unit Delay/1, pose/1
  Acceleration to Velocity/1 -> callPlatformDynamics/3(velocity), Velocity to Position/1  "rate"
  Unit Delay1/1 -> sat. forces/1
  Model Thrusters/1(forces) -> Unit Delay1/1, callPlatformDynamics/1(forces)
  duty/1 -> Model Thrusters/1(duty)
  Velocity to Position/1 -> callMeasureState/1(truePose), Model Thrusters/3(pose), callPlatformDynamics/2(position)  "pose"
  Unit Delay/1 -> callMeasureState/3(previousMeasured)
  callPlatformDynamics/1(acceleration) -> Acceleration to Velocity/1
  floating/1 -> callPlatformDynamics/4(floating)
  time/1 -> callMeasureState/2(time), Model Thrusters/2(time)

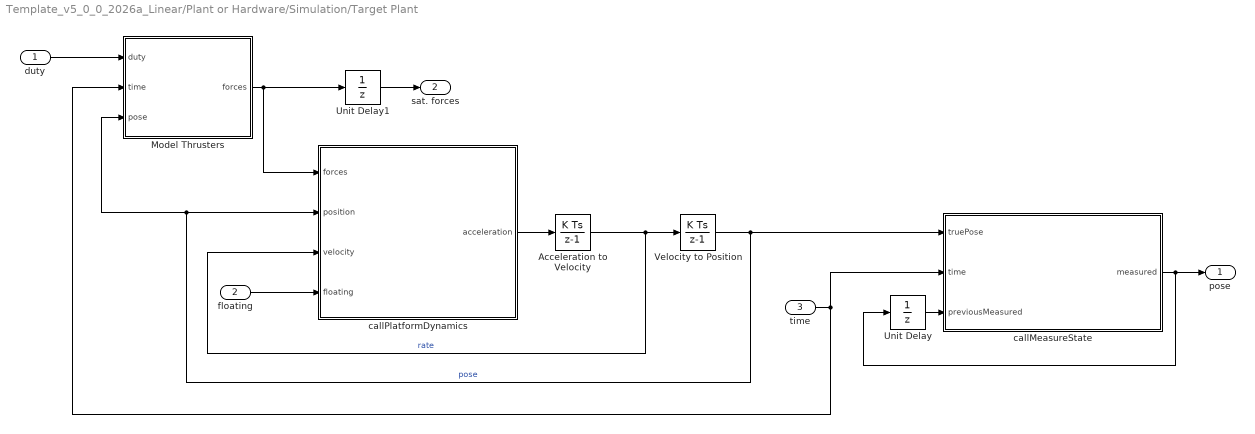
== system Template_v5_0_0_2026a_Linear/Plant or Hardware/Simulation/Target Plant ==
  duty : Inport
  floating : Inport  Port=2
  time : Inport  Port=3
  Acceleration to Velocity : DiscreteIntegrator  SampleTime=-1  ICPrevOutput=DiscIntNeverNeededParam  ICPrevScaledInput=DiscIntNeverNeededParam
  Model Thrusters : Subsystem
  Unit Delay : UnitDelay  SampleTime=-1
  Unit Delay1 : UnitDelay  SampleTime=-1
  Velocity to Position : DiscreteIntegrator  InitialCondition=initialPose  SampleTime=-1  ICPrevOutput=DiscIntNeverNeededParam  ICPrevScaledInput=DiscIntNeverNeededParam
  callMeasureState : MATLAB Function  TreatAsAtomicUnit=on
  callPlatformDynamics : MATLAB Function  TreatAsAtomicUnit=on
  pose : Outport
  sat. forces : Outport  Port=2
  wires:
  callMeasureState/1(measured) -> Unit Delay/1, pose/1
  Acceleration to Velocity/1 -> callPlatformDynamics/3(velocity), Velocity to Position/1  "rate"
  Unit Delay1/1 -> sat. forces/1
  Model Thrusters/1(forces) -> Unit Delay1/1, callPlatformDynamics/1(forces)
  duty/1 -> Model Thrusters/1(duty)
  Velocity to Position/1 -> callMeasureState/1(truePose), Model Thrusters/3(pose), callPlatformDynamics/2(position)  "pose"
  Unit Delay/1 -> callMeasureState/3(previousMeasured)
  callPlatformDynamics/1(acceleration) -> Acceleration to Velocity/1
  floating/1 -> callPlatformDynamics/4(floating)
  time/1 -> callMeasureState/2(time), Model Thrusters/2(time)

== system Template_v5_0_0_2026a_Linear/Plant or Hardware/Simulation/Chaser Plant/Model Thrusters ==
  duty : Inport
  time : Inport  Port=2
  pose : Inport  Port=3
  Unit Delay2 : UnitDelay  SampleTime=-1
  callHoldDuty : MATLAB Function  TreatAsAtomicUnit=on
  callThrusterForces : MATLAB Function  TreatAsAtomicUnit=on
  forces : Outport
  wires:
  Unit Delay2/1 -> callHoldDuty/2(previousDuty)
  callThrusterForces/1(forces) -> forces/1
  duty/1 -> callHoldDuty/1(newDuty)
  time/1 -> callHoldDuty/3(time)
  pose/1 -> callThrusterForces/2(pose)
  callHoldDuty/1(duty) -> Unit Delay2/1, callThrusterForces/1(duty)

== system Template_v5_0_0_2026a_Linear/Plant or Hardware/Simulation/Obstacle Plant/Model Thrusters ==
  duty : Inport
  time : Inport  Port=2
  pose : Inport  Port=3
  Unit Delay2 : UnitDelay  SampleTime=-1
  callHoldDuty : MATLAB Function  TreatAsAtomicUnit=on
  callThrusterForces : MATLAB Function  TreatAsAtomicUnit=on
  forces : Outport
  wires:
  Unit Delay2/1 -> callHoldDuty/2(previousDuty)
  callThrusterForces/1(forces) -> forces/1
  duty/1 -> callHoldDuty/1(newDuty)
  time/1 -> callHoldDuty/3(time)
  pose/1 -> callThrusterForces/2(pose)
  callHoldDuty/1(duty) -> Unit Delay2/1, callThrusterForces/1(duty)

== system Template_v5_0_0_2026a_Linear/Plant or Hardware/Simulation/Target Plant/Model Thrusters ==
  duty : Inport
  time : Inport  Port=2
  pose : Inport  Port=3
  Unit Delay2 : UnitDelay  SampleTime=-1
  callHoldDuty : MATLAB Function  TreatAsAtomicUnit=on
  callThrusterForces : MATLAB Function  TreatAsAtomicUnit=on
  forces : Outport
  wires:
  Unit Delay2/1 -> callHoldDuty/2(previousDuty)
  callThrusterForces/1(forces) -> forces/1
  duty/1 -> callHoldDuty/1(newDuty)
  time/1 -> callHoldDuty/3(time)
  pose/1 -> callThrusterForces/2(pose)
  callHoldDuty/1(duty) -> Unit Delay2/1, callThrusterForces/1(duty)

== matlab function Template_v5_0_0_2026a_Linear/Plant or Hardware/Simulation/Obstacle Plant/Model Thrusters/callHoldDuty ==
  data: duty output; newDuty input; previousDuty input; time input; PWMFreq parameter; baseRate parameter
function duty = callHoldDuty(newDuty, previousDuty, time, PWMFreq, baseRate)

    duty = spot.control.holdDuty(newDuty, previousDuty, time, PWMFreq, baseRate);

end

== matlab function Template_v5_0_0_2026a_Linear/Subsystem/Sample Chaser Experiment ==
  data: goal output; controllerChoice output; bus input; xLength parameter; yLength parameter; Phase2_End parameter; plannerChoice output
function [goal, controllerChoice, plannerChoice] = sampleChaserExperiment(bus, xLength, yLength, Phase2_End)
    %SAMPLECHASEREXPERIMENT Circle around the table centre.
    %   The goal moves at a constant angular rate around a circle at the table centre,
    %   starting when phase 3 starts, and the chaser faces outward along the radius.

    RADIUS = 0.85;              % [m]
    RATE   = 0.03490659;        % [rad/s] (2 deg/s)
    OFFSET = 0;                 % starting angle [rad] (v5: BLACK 2*pi/3, BLUE 4*pi/3)

    % Time since the experiment started, and where on the circle that puts the goal
    t     = bus.time - Phase2_End;      % [s]
    angle = RATE * t + OFFSET;          % [rad]

    goal = [xLength/2 + RADIUS * cos(angle);    % [m]
            yLength/2 + RADIUS * sin(angle);    % [m]
            atan2(sin(angle), cos(angle))];     % [rad], wrapped to [-pi, pi]

    controllerChoice = 1;       % default LQR
    plannerChoice    = 0;
end

== matlab function Template_v5_0_0_2026a_Linear/Subsystem/Sample Target Experiment ==
  data: goal output; controllerChoice output; bus input; xLength parameter; yLength parameter; Phase2_End parameter; plannerChoice output
function [goal, controllerChoice, plannerChoice] = sampleTargetExperiment(bus, xLength, yLength, Phase2_End)
    %SAMPLECHASEREXPERIMENT Circle around the table centre.
    %   The goal moves at a constant angular rate around a circle at the table centre,
    %   starting when phase 3 starts, and the chaser faces outward along the radius.

    RADIUS = 0.85;              % [m]
    RATE   = 0.03490659;        % [rad/s] (2 deg/s)
    OFFSET = 2*pi/3;                 % starting angle [rad] (v5: BLACK 2*pi/3, BLUE 4*pi/3)

    % Time since the experiment started, and where on the circle that puts the goal
    t     = bus.time - Phase2_End;      % [s]
    angle = RATE * t + OFFSET;          % [rad]

    goal = [xLength/2 + RADIUS * cos(angle);    % [m]
            yLength/2 + RADIUS * sin(angle);    % [m]
            atan2(sin(angle), cos(angle))];     % [rad], wrapped to [-pi, pi]

    controllerChoice = 1;       % default LQR
    plannerChoice    = 0;
end

== matlab function Template_v5_0_0_2026a_Linear/Subsystem/Sample Obstacle Experiment ==
  data: goal output; controllerChoice output; bus input; xLength parameter; yLength parameter; Phase2_End parameter; plannerChoice output
function [goal, controllerChoice, plannerChoice] = sampleTargetExperiment(bus, xLength, yLength, Phase2_End)
    %SAMPLECHASEREXPERIMENT Circle around the table centre.
    %   The goal moves at a constant angular rate around a circle at the table centre,
    %   starting when phase 3 starts, and the chaser faces outward along the radius.

    RADIUS = 0.85;              % [m]
    RATE   = 0.03490659;        % [rad/s] (2 deg/s)
    OFFSET = 4*pi/3;                 % starting angle [rad] (v5: BLACK 2*pi/3, BLUE 4*pi/3)

    % Time since the experiment started, and where on the circle that puts the goal
    t     = bus.time - Phase2_End;      % [s]
    angle = RATE * t + OFFSET;          % [rad]

    goal = [xLength/2 + RADIUS * cos(angle);    % [m]
            yLength/2 + RADIUS * sin(angle);    % [m]
            atan2(sin(angle), cos(angle))];     % [rad], wrapped to [-pi, pi]

    controllerChoice = 1;       % default LQR
    plannerChoice    = 0;
end

== matlab function Template_v5_0_0_2026a_Linear/Plant or Hardware/Simulation/MATLAB Function ==
  data: bus input Bus: SpotBus; packet output Bus: LogPacket
function packet = callLogPacket(bus)
    packet = spot.buses.logPacket(bus);
end

== matlab function Template_v5_0_0_2026a_Linear/Path Planners/Target Planner/callPlanner ==
  data: plannerChoice input; state input Bus: PlatformState; setpoint output Bus: Setpoint; goal input; previousGoal input; context input; maxSpeed parameter; maxTurnRate parameter; horizon parameter; customParams parameter; baseRate parameter
function setpoint = callPlanner(plannerChoice, state, goal, previousGoal, context, maxSpeed, maxTurnRate, horizon, customParams, baseRate)
    %CALLPLANNER Run the selected path planner for one spacecraft.
    %   plannerChoice  0 none (the goal is the setpoint), 1 default, 2 custom,
    %                  anything else hold the current pose

    switch plannerChoice
        case 0
            setpoint = spot.guidance.directPlanner(goal, previousGoal, baseRate);
        case 1
            setpoint = spot.guidance.defaultPlanner(state, goal, maxSpeed, maxTurnRate, horizon);
        case 2
            setpoint = spot.guidance.customPlanner(state, goal, context, customParams);
        otherwise
            setpoint.pose = state.pose;         % hold where it is
            setpoint.rate = zeros(3, 1);
    end
end

== matlab function Template_v5_0_0_2026a_Linear/Path Planners/Obstacle Planner/callPlanner ==
  data: plannerChoice input; state input Bus: PlatformState; setpoint output Bus: Setpoint; goal input; previousGoal input; context input; maxSpeed parameter; maxTurnRate parameter; horizon parameter; customParams parameter; baseRate parameter
function setpoint = callPlanner(plannerChoice, state, goal, previousGoal, context, maxSpeed, maxTurnRate, horizon, customParams, baseRate)
    %CALLPLANNER Run the selected path planner for one spacecraft.
    %   plannerChoice  0 none (the goal is the setpoint), 1 default, 2 custom,
    %                  anything else hold the current pose

    switch plannerChoice
        case 0
            setpoint = spot.guidance.directPlanner(goal, previousGoal, baseRate);
        case 1
            setpoint = spot.guidance.defaultPlanner(state, goal, maxSpeed, maxTurnRate, horizon);
        case 2
            setpoint = spot.guidance.customPlanner(state, goal, context, customParams);
        otherwise
            setpoint.pose = state.pose;         % hold where it is
            setpoint.rate = zeros(3, 1);
    end
end

== matlab function Template_v5_0_0_2026a_Linear/Plant or Hardware/Simulation/Chaser Plant/Model Thrusters/callHoldDuty ==
  data: duty output; newDuty input; previousDuty input; time input; PWMFreq parameter; baseRate parameter
function duty = callHoldDuty(newDuty, previousDuty, time, PWMFreq, baseRate)

    duty = spot.control.holdDuty(newDuty, previousDuty, time, PWMFreq, baseRate);

end

== matlab function Template_v5_0_0_2026a_Linear/Plant or Hardware/Simulation/Target Plant/callPlatformDynamics ==
  data: forces input; position input; velocity input; floating input; acceleration output; mass parameter; inertia parameter; tableSlope parameter; tableDamping parameter
function acceleration  = callPlatformDynamics(forces, position, velocity,...
    floating, mass, inertia, tableSlope, tableDamping)

    [acceleration] = spot.dynamics.platformDynamics(forces, position,...
        velocity, floating, mass, inertia, tableSlope, tableDamping);
    
end

== matlab function Template_v5_0_0_2026a_Linear/Plant or Hardware/Simulation/Obstacle Plant/Model Thrusters/callThrusterForces ==
  data: duty input; pose input; thrusterDist parameter; thrust parameter; forces output; decayPerValve parameter
function forces = callThrusterForces(duty, pose, thrusterDist, thrust, decayPerValve)

    forces = spot.dynamics.thrusterForces(duty, pose(3), thrusterDist, thrust, decayPerValve);

end

== matlab function Template_v5_0_0_2026a_Linear/Plant or Hardware/Simulation/Chaser Plant/callMeasureState ==
  data: truePose input; time input; measured output Bus: PlatformState; previousMeasured input Bus: PlatformState; dataRate parameter; baseRate parameter
function measured = callMeasureState(truePose, time, previousMeasured, dataRate, baseRate)

    measured = spot.dynamics.measureState(truePose, previousMeasured, time, dataRate, baseRate);

end

== matlab function Template_v5_0_0_2026a_Linear/Plant or Hardware/Simulation/Obstacle Plant/callMeasureState ==
  data: truePose input; time input; measured output Bus: PlatformState; previousMeasured input Bus: PlatformState; dataRate parameter; baseRate parameter
function measured = callMeasureState(truePose, time, previousMeasured, dataRate, baseRate)

    measured = spot.dynamics.measureState(truePose, previousMeasured, time, dataRate, baseRate);

end

== matlab function Template_v5_0_0_2026a_Linear/Controllers/Target Controller/callController ==
  data: controllerChoice input; state input; setpoint input; controls output; context input Bus: SpotBus; K parameter; customParams parameter
function controls = callController(controllerChoice, state, setpoint, context, K, customParams)
    %CALLCONTROLLER Run the selected control law for one spacecraft.
    %   controllerChoice  1 default LQR, 2 custom, anything else thrusters off
    
    switch controllerChoice
        case 1
            controls = spot.control.defaultController(state, setpoint, K);
        case 2
            controls = spot.control.customController(state, setpoint, context, customParams);
        otherwise
            controls = zeros(3, 1);     % thrusters off
    end
end

== matlab function Template_v5_0_0_2026a_Linear/Plant or Hardware/Simulation/Obstacle Plant/callPlatformDynamics ==
  data: forces input; position input; velocity input; floating input; acceleration output; mass parameter; inertia parameter; tableSlope parameter; tableDamping parameter
function acceleration  = callPlatformDynamics(forces, position, velocity,...
    floating, mass, inertia, tableSlope, tableDamping)

    [acceleration] = spot.dynamics.platformDynamics(forces, position,...
        velocity, floating, mass, inertia, tableSlope, tableDamping);
    
end

== matlab function Template_v5_0_0_2026a_Linear/Plant or Hardware/Experiment/Call Send Experiment Time ==
  data: t input; whoAmI input; labConsoleIP parameter
function callSendExperimentTime(t, whoAmI, labConsoleIP)

    spot.hardware.sendExperimentTime(t, whoAmI, labConsoleIP);

end

== matlab function Template_v5_0_0_2026a_Linear/Plant or Hardware/Experiment/Call Thruster Command ==
  data: bus input Bus: SpotBus; frame output uint8 size=[37 1]; whoAmI input
function frame = callThrusterCommand(bus, whoAmI)

    frame = spot.hardware.thrusterCommand(bus, whoAmI);

end

== matlab function Template_v5_0_0_2026a_Linear/Plant or Hardware/Experiment/States and Experiment Time ==
  data: t output; packet input; red output Bus: PlatformState; black output Bus: PlatformState; blue output Bus: PlatformState; age input
function [t, red, black, blue] = callPhaseSpaceStates(packet, age)

    [t, ~] = spot.hardware.experimentTime(packet, age);
    [red, black, blue] = spot.hardware.phaseSpaceStates(packet);

end

== matlab function Template_v5_0_0_2026a_Linear/Plant or Hardware/Experiment/Call Log Vector ==
  data: bus input Bus: SpotBus; values output; count output
function [values, count] = callLogVector(bus)

    [values, count] = spot.hardware.logVector(spot.buses.logPacket(bus));

end

== matlab function Template_v5_0_0_2026a_Linear/Plant or Hardware/Experiment/Receive PhaseSpace Data ==
  data: packet output; newPackets output; age output; labConsoleIP parameter
function [packet, newPackets, age] = receivePhaseSpaceData(labConsoleIP)
%RECEIVEPHASESPACEDATA The newest PhaseSpace packet from the lab console (TX2), every step.
%   packet: 115 values (positions, velocities, LEDs and, during an experiment, the experiment
%   clock); newPackets: packets since the last step; age: seconds since it arrived (-1 = none
%   yet). See help spot.hardware.phasespaceLatest.
%#codegen
[packet, newPackets, age] = spot.hardware.phasespaceLatest(31534, labConsoleIP);
end
